simulink model "Pulse_Sweep_Model_Snapshot"  (R2026a)
settings: Solver=ode15s  StopTime=10  MaxStep=0.001  RelTol=1e-8  AbsTol=1e-10
model workspace (MAT data in the model file):
  K_lqr_controller = [-0.00284705017361 0.122689000645 -0.00232682606921 0.00886461536906]
  K_pp_controller = [-0.00262883953839 0.104642532618 -0.00218085328178 0.00778047678221]
  pid_ArmD = 0.00283510926632
  pid_ArmI = 0.0007
  pid_ArmP = 0.00184018767687
  pid_Kaw = 20
  pid_PendD = 0.00972559597776
  pid_PendP = 0.104642532618
  smiData.RigidTransform(1).translation = [-244.660692531 -37.8098812469 -477.156945201]
  smiData.RigidTransform(1).angle = 2.55760922614
  smiData.RigidTransform(1).axis = [0.300426658947 0.67440706052 0.674476789308]
  smiData.RigidTransform(1).ID = "B[modern conttrol_Pendulum .stp-1:-:modern conttrol_ horizontal_arm .stp-1]"
  smiData.RigidTransform(2).translation = [-247.634754981 -40.4847554626 -477.157635298]
  smiData.RigidTransform(2).angle = 2.55760922614
  smiData.RigidTransform(2).axis = [0.300426658947 0.67440706052 0.674476789308]
  smiData.RigidTransform(2).ID = "F[modern conttrol_Pendulum .stp-1:-:modern conttrol_ horizontal_arm .stp-1]"
  smiData.RigidTransform(3).translation = [-272.175879601 -62.5545266142 -447.163329111]
  smiData.RigidTransform(3).angle = 3.14152402451
  smiData.RigidTransform(3).axis = [-0.999999996374 2.92211836945e-09 -8.51568583922e-05]
  smiData.RigidTransform(3).ID = "B[modern conttrol_ horizontal_arm .stp-1:-:modern conttrol_ BASE .stp-1]"
  smiData.RigidTransform(4).translation = [-272.175879601 -62.5545266142 -447.163329111]
  smiData.RigidTransform(4).angle = 3.14152402451
  smiData.RigidTransform(4).axis = [-0.999999996374 2.92211836944e-09 -8.51568583922e-05]
  smiData.RigidTransform(4).ID = "F[modern conttrol_ horizontal_arm .stp-1:-:modern conttrol_ BASE .stp-1]"
  smiData.RigidTransform(5).translation = [-901.384854799 -324.852677228 2108.86942688]
  smiData.RigidTransform(5).angle = 2.09421753207
  smiData.RigidTransform(5).axis = [0.577330696727 -0.577330696727 0.577389412124]
  smiData.RigidTransform(5).ID = "RootGround[modern conttrol_ BASE .stp-1]"
  smiData.Solid(1).mass = 0.183317957018
  smiData.Solid(1).CoM = [-10.7361053602 -2.48129316166 -18.6438450111]
  smiData.Solid(1).MoI = [0.234552178635 0.234414857876 0.220551589316]
  smiData.Solid(1).PoI = [-0.000864428028976 -0.000962178736372 0.000630134655694]
  smiData.Solid(1).color = [0.745098039216 0.737254901961 0.729411764706]
  smiData.Solid(1).opacity = 1
  smiData.Solid(1).ID = "modern conttrol_ horizontal_arm .stp*:*Default"
  smiData.Solid(2).mass = 0.00722125286234
  smiData.Solid(2).CoM = [-8.92893482987 -1.82055355389 -18.2809598406]
  smiData.Solid(2).MoI = [0.0072083021969 0.0106803033814 0.00963261515156]
  smiData.Solid(2).PoI = [0.00327189358985 -0.00494008093961 0.00363251936408]
  smiData.Solid(2).color = [0.894117647059 0.894117647059 0.894117647059]
  smiData.Solid(2).opacity = 1
  smiData.Solid(2).ID = "modern conttrol_Pendulum .stp*:*Default"
  smiData.Solid(3).mass = 0.277142549471
  smiData.Solid(3).CoM = [-10.7265338957 -2.42898357651 -14.4295668435]
  smiData.Solid(3).MoI = [0.902926430859 0.896181432603 0.660496847328]
  smiData.Solid(3).PoI = [-0.0116443332078 0.00507741067153 0.00049862544881]
  smiData.Solid(3).color = [0.745098039216 0.737254901961 0.729411764706]
  smiData.Solid(3).opacity = 1
  smiData.Solid(3).ID = "modern conttrol_ BASE .stp*:*Default"
  smiData.RevoluteJoint(1).Rz.Pos = -7.13735250286e-12
  smiData.RevoluteJoint(1).ID = "[modern conttrol_Pendulum .stp-1:-:modern conttrol_ horizontal_arm .stp-1]"
  smiData.RevoluteJoint(2).Rz.Pos = -14.9000381004
  smiData.RevoluteJoint(2).ID = "[modern conttrol_ horizontal_arm .stp-1:-:modern conttrol_ BASE .stp-1]"
  tau_limit_sim = 0.01
  taue_controller = 6.71011527243e-16
  xe_controller = [0; 3.17402050778e-05; 0; 0]
undefined symbols (not defined in the file or in its folder): X, Y, Z
libraries: sm_lib x15, nesl_utility x6
settings Model: Creator=youss  LastModifiedBy=youss
settings ExplorerConfigSet: InternalSimMechanicsExplorerSettings=|
  | <ExplorerConfiguration>
  | 
  |   <canonicalview>planar_xy</canonicalview>
  | 
  |   <TilePanel>
  |     <TileInfo>
  |       <Tiles Columns="1" Count="1" Height="661" Rows="1" Width="1082">
  |         <Row Weight="1"/>
  |         <Column Weight="1"/>
  |         <Tile Height="1" Width="1" X="0" Y="0"/>
  |       </Tiles>
  |     </TileInfo>
  |     <SceneInfo>
  |       <SceneViewer>
  |         <IsThisViewStd>
  |           <IsStandardView>off</IsStandardView>
  |           <StandardViewName>Front</StandardViewName>
  |         </IsThisViewStd>
  |         <BGColor>
  |           <R>1</R>
  |           <G>1</G>
  |           <B>1</B>
  |           <A>1</A>
  |         </BGColor>
  |         <Camera>
  |           <DoPerspective>off</DoPerspective>
  |           <Position>
  |             <X>-0.83937932035154528</X>
  |             <Y>0.78777288036255699</Y>
  |             <Z>2.49476630807056</Z>
  |           </Position>
  |           <Center>
  |             <X>-0.83937932035154528</X>
  |             <Y>0.12962840465429493</Y>
  |             <Z>1.8366218323622983</Z>
  |           </Center>
  |           <Up>
  |             <X>0</X>
  |             <Y>0.70710678118654735</Y>
  |             <Z>-0.70710678118654768</Z>
  |           </Up>
  |           <XLim>0.13809857222982996</XLim>
  |           <YLim>0.13809857222982996</YLim>
  |           <ViewLimDist>0.01</ViewLimDist>
  |         </Camera>
  |       </SceneViewer>
  |     </SceneInfo>
  |   </TilePanel>
  | 
  |   <MechEditorPanel>
  |     <GfxPanelCameraMap/>
  |     <Cameras/>
  |     <VideoCreator>
  |       <IncludeTiles>All</IncludeTiles>
  |       <IncludeTime>on</IncludeTime>
  |       <IncludeWorldFrame>off</IncludeWorldFrame>
  |       <PlaybackSpeedRatio>1</PlaybackSpeedRatio>
  |       <FrameRate>30</FrameRate>
  |       <FrameSize>auto</FrameSize>
  |       <VideoFormat>UncompressedAVI</VideoFormat>
  |     </VideoCreator>
  |   </MechEditorPanel>
  | 
  |   <PlaybackSettings>
  |     <PlaybackSpeedFactor>1</PlaybackSpeedFactor>
  |   </PlaybackSettings>
  | 
  | </ExplorerConfiguration>

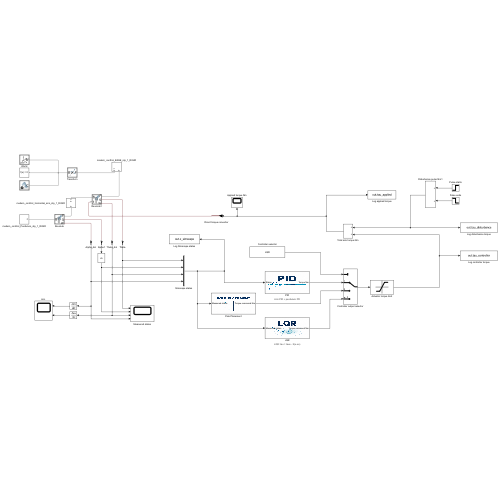
[thumbnail: Simulink's stored preview of the top-level diagram]
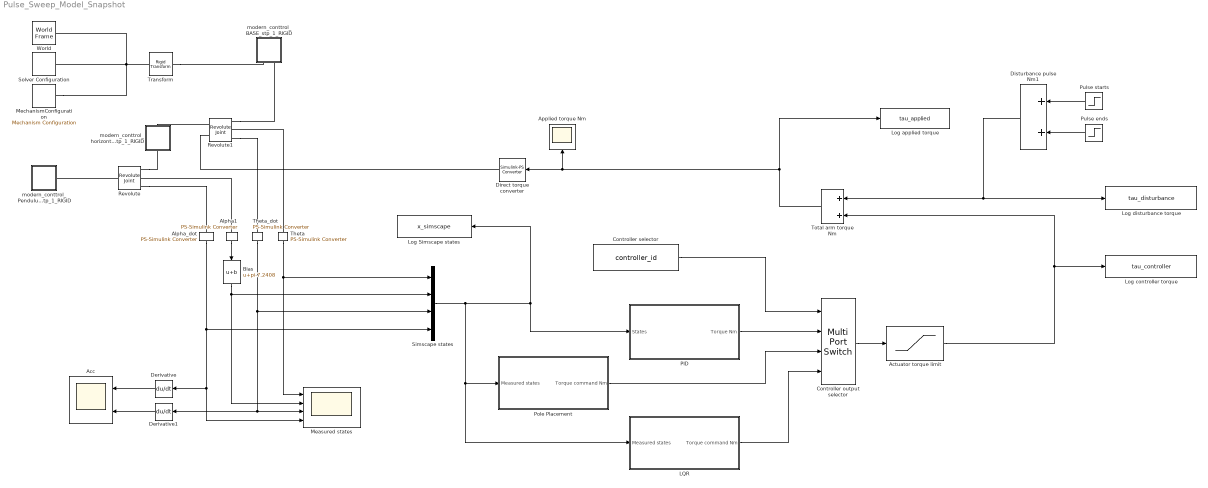
== system Pulse_Sweep_Model_Snapshot ==
  "Acc " : Scope  NumInputPorts=2
      settings: ActiveDisplayYMinimum=-146.28941148090837  ActiveDisplayYMaximum=145.24989573549755  YLabel=Arm
  Actuator torque limit : Saturate  UpperLimit=tau_limit_sim  LowerLimit=-tau_limit_sim
  Alpha1 : nesl_utility/PS-Simulink Converter  PhysicalDomain=network_engine_domain  SubClassName=ps_output  LeftPortType=input  RightPortType=output  PseudoPeriodic=off  Frequencies=[]  VectorFormat=inherit  Unit=rad  AffineConversion=off
  Alpha_dot : nesl_utility/PS-Simulink Converter  PhysicalDomain=network_engine_domain  SubClassName=ps_output  LeftPortType=input  RightPortType=output  PseudoPeriodic=off  Frequencies=[]  VectorFormat=inherit  Unit=rad/s  AffineConversion=off
  Applied torque Nm : Scope
      settings: Title=Total applied arm torque  ActiveDisplayYMinimum=-0.012433392383790797  ActiveDisplayYMaximum=0.014826694316528995  YLabel=N m
  Bias : Bias  Bias=pi-7.2408  SaturateOnIntegerOverflow=off
  Controller output selector : MultiPortSwitch  SaturateOnIntegerOverflow=off  InputSameDT=off
  Controller selector : Constant  Value=controller_id  SampleTime=0  mask{controller_choice=LQR}
      mask prompts: controller_choice "Controller"
      mask help: Choose the controller before simulation. PID and LQR are reserved until their gains are designed.
      mask init:
      | controller_id=find(strcmp(controller_choice,{'PID','Pole Placement','LQR'}));
      mask TypeOptions controller_choice: PID | Pole Placement | LQR
      mask Display: disp(controller_choice)
  Derivative : Derivative
  Derivative1 : Derivative
  Direct torque converter : nesl_utility/Simulink-PS Converter  PhysicalDomain=network_engine_domain  SubClassName=ps_input  LeftPortType=input  RightPortType=output  PseudoPeriodic=off  Frequencies=[]  NoiseDistribution=none  NoiseParameters=[]  Unit=N*m  AffineConversion=off  FilteringAndDerivatives=provide  SimscapeFilterOrder=1  InputFilterTimeConstant=0.001  UdotUserProvided=0
  Disturbance pulse Nm1 : Sum
  LQR : Subsystem  Description=Continuous four-state LQR using measured Multibody states. Shared actuator saturation remains outside the controller.
      settings: AttributesFormatString=LQR: tau = taue - K(x-xe)
      mask Display: image('ChatGPT Image Oct 27, 2026, 06_34_36 PM.png');
  Log Simscape states : ToWorkspace  VariableName=x_simscape  SaveFormat=Timeseries  SampleTime=-1
  Log applied torque : ToWorkspace  VariableName=tau_applied  SaveFormat=Timeseries  SampleTime=-1
  Log controller torque : ToWorkspace  VariableName=tau_controller  SaveFormat=Timeseries  SampleTime=-1
  Log disturbance torque : ToWorkspace  VariableName=tau_disturbance  SaveFormat=Timeseries  SampleTime=-1
  Measured states : Scope  NumInputPorts=4
      settings: Title=Arm angle - theta  ActiveDisplayYMinimum=-0.33373854489322996  ActiveDisplayYMaximum=0.16467513422765392  YLabel=rad
  MechanismConfiguration : sm_lib/Utilities/Mechanism Configuration  UniformGravity=Constant  GravityVector=[0 -9.81 0]  GravityVectorUnits=m/s^2  LinearizationDelta=0.001  JointModeTransitionNonlinearIterations=2
  PID : Subsystem  Description=Simple P/I/D paths. Select controller before each fresh run. No inactive tracking or live switching.
      settings: AttributesFormatString=Arm PID + pendulum PD
      mask Display: image('ChatGPT Image Oct 27, 2026, 06_33_53 PM.png');
  Pole Placement : Subsystem
      mask Display: image('ChatGPT Image Oct 27, 2026, 06_34_26 PM.png');
  Pulse ends : Step  Time=1.05  FinalValue=-0.01  SampleTime=0
  Pulse starts : Step  FinalValue=0.01  SampleTime=0
  Revolute : sm_lib/Joints/Revolute Joint  JointMode=Normal  CompositeWrenchDir=FollowerOnBase  CompositeWrenchFrame=BaseFrame  SenseConstraintForce=off  SenseConstraintTorque=off  SenseTotalForce=off  SenseTotalTorque=off  PositionTargetSpecify=on  PositionTargetPriority=High  PositionTargetValue=7.2408 -pi  PositionTargetValueUnits=rad  VelocityTargetSpecify=on  VelocityTargetPriority=High  VelocityTargetValue=0  VelocityTargetValueUnits=rad/s  EquilibriumPosition=0  EquilibriumPositionUnits=deg  SpringStiffness=0  SpringStiffnessUnits=N*m/deg  DampingCoefficient=5.5e-7  DampingCoefficientUnits=N*m/(deg/s)  LowerLimitSpecify=off  LowerLimitBound=-90  LowerLimitBoundUnits=deg  LowerLimitStiffness=1e4  LowerLimitStiffnessUnits=N*m/deg  LowerLimitDamping=10  LowerLimitDampingUnits=N*m/(deg/s)  LowerLimitTransitionRegionWidth=0.1  LowerLimitTransitionRegionWidthUnits=deg  UpperLimitSpecify=off  UpperLimitBound=90  UpperLimitBoundUnits=deg  UpperLimitStiffness=1e4  UpperLimitStiffnessUnits=N*m/deg  UpperLimitDamping=10  UpperLimitDampingUnits=N*m/(deg/s)  UpperLimitTransitionRegionWidth=0.1  UpperLimitTransitionRegionWidthUnits=deg  TorqueActuationMode=NoTorque  MotionActuationMode=ComputedMotion  SensePosition=on  SenseVelocity=on  SenseAcceleration=off  SenseTorqueForce=off  SenseLowerLimitTorqueForce=off  SenseUpperLimitTorqueForce=off
  Revolute1 : sm_lib/Joints/Revolute Joint  JointMode=Normal  CompositeWrenchDir=FollowerOnBase  CompositeWrenchFrame=BaseFrame  SenseConstraintForce=off  SenseConstraintTorque=off  SenseTotalForce=off  SenseTotalTorque=off  PositionTargetSpecify=off  PositionTargetPriority=High  PositionTargetValue=0  PositionTargetValueUnits=deg  VelocityTargetSpecify=off  VelocityTargetPriority=High  VelocityTargetValue=0  VelocityTargetValueUnits=deg/s  EquilibriumPosition=0  EquilibriumPositionUnits=deg  SpringStiffness=0  SpringStiffnessUnits=N*m/deg  DampingCoefficient=1e-5  DampingCoefficientUnits=N*m/(deg/s)  LowerLimitSpecify=off  LowerLimitBound=-90  LowerLimitBoundUnits=deg  LowerLimitStiffness=1e4  LowerLimitStiffnessUnits=N*m/deg  LowerLimitDamping=10  LowerLimitDampingUnits=N*m/(deg/s)  LowerLimitTransitionRegionWidth=0.1  LowerLimitTransitionRegionWidthUnits=deg  UpperLimitSpecify=off  UpperLimitBound=90  UpperLimitBoundUnits=deg  UpperLimitStiffness=1e4  UpperLimitStiffnessUnits=N*m/deg  UpperLimitDamping=10  UpperLimitDampingUnits=N*m/(deg/s)  UpperLimitTransitionRegionWidth=0.1  UpperLimitTransitionRegionWidthUnits=deg  TorqueActuationMode=InputTorque  MotionActuationMode=ComputedMotion  SensePosition=on  SenseVelocity=on  SenseAcceleration=off  SenseTorqueForce=off  SenseLowerLimitTorqueForce=off  SenseUpperLimitTorqueForce=off
  Simscape states : Mux
  Solver Configuration : nesl_utility/Solver Configuration  PhysicalDomain=network_engine_domain  SubClassName=solver  LeftPortType=input  RightPortType=generic  Tones=[]  Harmonics=[]  SimulateNoise=off  Profile=off  UseLocalSampling=off  EnableSwitchedLinearOptims=on  FrequencyDomain=off  UseCCode=off  RelTol=0.001  AbsTol=0.001  MinStep=1e-09  ToWorkspace=off  RevertToSquareIcSolve=off  NumHomotopyIterations=100  PhasorMode=off  PhasorModeNumHarmonics=1  ConsistencySolver=NEWTON_XTOL_AFTER_FTOL  CanonicalOrdering=CANONICAL  OptimizeIntermediates=OPTIMIZED  IndexReductionMethod=DerivativeReplacement  DoDC=off  ResidualTolerance=1e-09  ConsistencyTolSource=GLOBAL  ConsistencyAbsTol=0.001  ConsistencyRelTol=0.001  ConsistencyTolFactor=0.001  UseLocalSolver=off  LocalSolverChoice=NE_BACKWARD_EULER_ADVANCER  ResolveIndetEquations=on  FunctionEvalNumThread=1  LocalSolverSampleTime=0.001  DoFixedCost=off  MaxNonlinIter=3  MaxModeIter=2  ComputeImpulses=off  ImpulseIterations=2  LinearAlgebra=auto  LinearAlgebraNumThread=0  EquationFormulation=NE_TIME_EF  DelaysMemoryBudget=1024  AutomaticFiltering=on  FilteringTimeConstant=0.001  PartitionStorageMethod=AS_NEEDED  PartitionMemoryBudget=1024  PartitionMethod=ROBUST  MultibodyUseLocalSolver=off  MultibodyLocalSolverChoice=ODE1  MultibodyLocalSolverSampleTime=0.001
  Theta : nesl_utility/PS-Simulink Converter  PhysicalDomain=network_engine_domain  SubClassName=ps_output  LeftPortType=input  RightPortType=output  PseudoPeriodic=off  Frequencies=[]  VectorFormat=inherit  Unit=rad  AffineConversion=off
  Theta_dot : nesl_utility/PS-Simulink Converter  PhysicalDomain=network_engine_domain  SubClassName=ps_output  LeftPortType=input  RightPortType=output  PseudoPeriodic=off  Frequencies=[]  VectorFormat=inherit  Unit=rad/s  AffineConversion=off
  Total arm torque Nm : Sum
  Transform : sm_lib/Frames and Transforms/Rigid Transform  RotationMethod=ArbitraryAxis  FollAlignAxisA=+X  BaseAlignAxisA=+Y  FollAlignAxisB=+Y  BaseAlignAxisB=+Z  RotationStandardAxis=+Z  RotationAngle=smiData.RigidTransform(5).angle  RotationAngleUnits=rad  RotationArbitraryAxis=smiData.RigidTransform(5).axis  RotationSequenceAxes=FollowerAxes  RotationSequence=XYX  RotationSequenceAngles=[0 0 0]  RotationSequenceAnglesUnits=deg  RotationMatrix=[1 0 0;0 1 0;0 0 1]  Quaternion=[1 0 0 0]  TranslationMethod=Cartesian  TranslationCartesianOffset=smiData.RigidTransform(5).translation  TranslationCartesianOffsetUnits=mm  TranslationStandardAxis=+Z  TranslationStandardOffset=0  TranslationStandardOffsetUnits=m  TranslationROffset=0  TranslationROffsetUnits=m  TranslationThetaOffset=0  TranslationThetaOffsetUnits=deg  TranslationZOffset=0  TranslationZOffsetUnits=m
  World : sm_lib/Frames and Transforms/World Frame
  modern_conttrol_BASE_stp_1_RIGID : Subsystem
  modern_conttrol_Pendulum_stp_1_RIGID : Subsystem
  modern_conttrol_horizontal_arm_stp_1_RIGID : Subsystem
  wires:
  Theta/1 -> Simscape states/1, Measured states/1
  Bias/1 -> Simscape states/2, Measured states/2
  Alpha1/1 -> Bias/1
  Simscape states/1 -> PID/1(States), Log Simscape states/1, LQR/1(Measured states), Pole Placement/1(Measured states)
  Total arm torque Nm/1 -> Applied torque Nm/1, Direct torque converter/1, Log applied torque/1
  Actuator torque limit/1 -> Total arm torque Nm/2, Log controller torque/1
  Controller selector/1 -> Controller output selector/1
  Pole Placement/1(Torque command Nm) -> Controller output selector/3
  LQR/1(Torque command Nm) -> Controller output selector/4
  Controller output selector/1 -> Actuator torque limit/1
  PID/1(Torque Nm) -> Controller output selector/2
  Derivative1/1 -> "Acc "/2
  Alpha_dot/1 -> Simscape states/4, Derivative/1, Measured states/4
  Derivative/1 -> "Acc "/1
  Theta_dot/1 -> Simscape states/3, Measured states/3, Derivative1/1
  Pulse ends/1 -> Disturbance pulse Nm1/2
  Pulse starts/1 -> Disturbance pulse Nm1/1
  Disturbance pulse Nm1/1 -> Log disturbance torque/1, Total arm torque Nm/1
  connections:
  MechanismConfiguration/RConn1 -- Transform/LConn1 -- Solver Configuration/RConn1 -- World/RConn1
  Revolute/LConn1 -- modern_conttrol_Pendulum_stp_1_RIGID/RConn1
  Revolute/RConn1 -- modern_conttrol_horizontal_arm_stp_1_RIGID/LConn1
  Revolute1/LConn1 -- modern_conttrol_horizontal_arm_stp_1_RIGID/RConn1
  Revolute1/RConn1 -- modern_conttrol_BASE_stp_1_RIGID/LConn2
  Transform/RConn1 -- modern_conttrol_BASE_stp_1_RIGID/LConn1
  Theta/LConn1 -- Revolute1/RConn2
  Revolute/RConn3 -- Alpha_dot/LConn1
  Alpha1/LConn1 -- Revolute/RConn2
  Revolute1/RConn3 -- Theta_dot/LConn1
  Direct torque converter/RConn1 -- Revolute1/LConn2

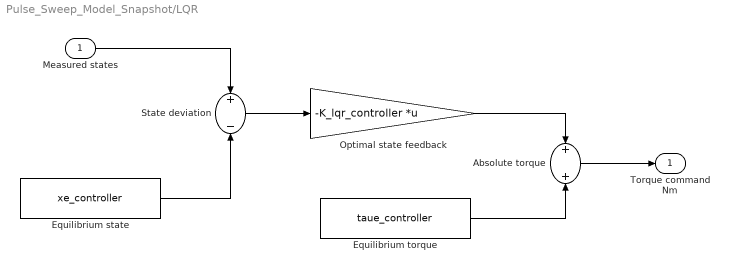
== system Pulse_Sweep_Model_Snapshot/LQR ==
  Measured states : Inport
  Absolute torque : Sum
  Equilibrium state : Constant  Value=xe_controller
  Equilibrium torque : Constant  Value=taue_controller
  Optimal state feedback : Gain  Gain=-K_lqr_controller  Multiplication=Matrix(K*u)
  State deviation : Sum  Inputs=+-
  Torque command Nm : Outport
  wires:
  Measured states/1 -> State deviation/1
  Equilibrium state/1 -> State deviation/2
  State deviation/1 -> Optimal state feedback/1
  Optimal state feedback/1 -> Absolute torque/1
  Equilibrium torque/1 -> Absolute torque/2
  Absolute torque/1 -> Torque command Nm/1

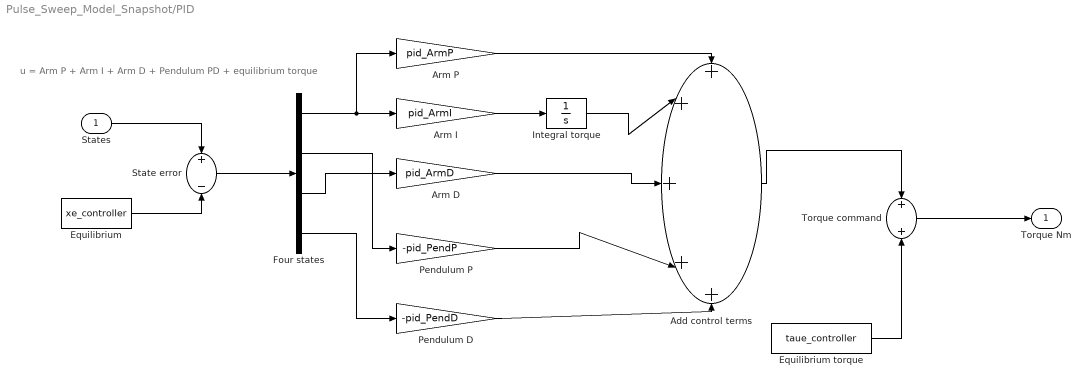
== system Pulse_Sweep_Model_Snapshot/PID ==
  note: u = Arm P + Arm I + Arm D + Pendulum PD + equilibrium torque
  States : Inport
  Add control terms : Sum  Inputs=+++++
  Arm D : Gain  Gain=pid_ArmD
  Arm I : Gain  Gain=pid_ArmI
  Arm P : Gain  Gain=pid_ArmP
  Equilibrium : Constant  Value=xe_controller
  Equilibrium torque : Constant  Value=taue_controller
  Four states : Demux
  Integral torque : Integrator  LimitOutput=on  UpperSaturationLimit=0.002  LowerSaturationLimit=-0.002
  Pendulum D : Gain  Gain=-pid_PendD
  Pendulum P : Gain  Gain=-pid_PendP
  State error : Sum  Inputs=+-
  Torque command : Sum
  Torque Nm : Outport
  wires:
  States/1 -> State error/1
  Equilibrium/1 -> State error/2
  State error/1 -> Four states/1
  Four states/1 -> Arm P/1, Arm I/1
  Four states/3 -> Arm D/1
  Four states/2 -> Pendulum P/1
  Four states/4 -> Pendulum D/1
  Arm I/1 -> Integral torque/1
  Arm P/1 -> Add control terms/1
  Integral torque/1 -> Add control terms/2
  Arm D/1 -> Add control terms/3
  Pendulum P/1 -> Add control terms/4
  Pendulum D/1 -> Add control terms/5
  Add control terms/1 -> Torque command/1
  Equilibrium torque/1 -> Torque command/2
  Torque command/1 -> Torque Nm/1

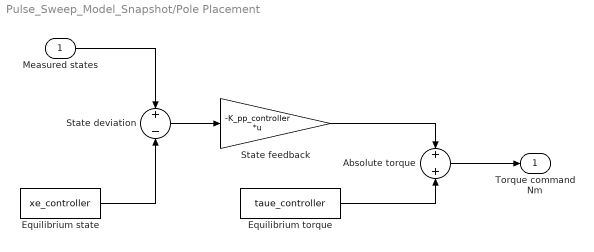
== system Pulse_Sweep_Model_Snapshot/Pole Placement ==
  Measured states : Inport
  Absolute torque : Sum
  Equilibrium state : Constant  Value=xe_controller
  Equilibrium torque : Constant  Value=taue_controller
  State deviation : Sum  Inputs=+-
  State feedback : Gain  Gain=-K_pp_controller  Multiplication=Matrix(K*u)
  Torque command Nm : Outport
  wires:
  Measured states/1 -> State deviation/1
  Equilibrium state/1 -> State deviation/2
  State deviation/1 -> State feedback/1
  State feedback/1 -> Absolute torque/1
  Equilibrium torque/1 -> Absolute torque/2
  Absolute torque/1 -> Torque command Nm/1

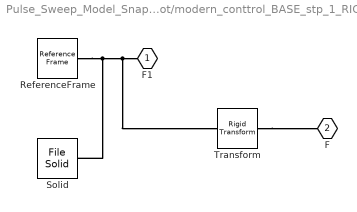
== system Pulse_Sweep_Model_Snapshot/modern_conttrol_BASE_stp_1_RIGID ==
  ReferenceFrame : sm_lib/Frames and Transforms/Reference Frame
  Solid : sm_lib/Body Elements/File Solid  ExtGeomFileName=modern conttrol_ BASE .stp_Default_sldprt.STEP  UnitType=FromFile  ExtGeomFileUnits=m  StepReaderType=HEX  ExportConvexHullGeometry=off  InertiaType=Custom  BasedOnType=DensityFromFile  Density=1000  DensityUnits=kg/m^3  Mass=smiData.Solid(3).mass  MassUnits=kg  CenterOfMass=smiData.Solid(3).CoM  CenterOfMassUnits=in  MomentsOfInertia=smiData.Solid(3).MoI  MomentsOfInertiaUnits=kg*in^2  ProductsOfInertia=smiData.Solid(3).PoI  ProductsOfInertiaUnits=kg*in^2  GraphicType=FromGeometry  MarkerShape=Sphere  MarkerSize=10  GraphicVisPropType=SimpleVisualProperties  GraphicDiffuseColor=[0.8745 0 0]  GraphicOpacity=smiData.Solid(3).opacity  GraphicSpecularColor=[0.5 0.5 0.5 1.0]  GraphicAmbientColor=[0.15 0.15 0.15 1.0]  GraphicEmissiveColor=[0.0 0.0 0.0 1.0]  GraphicShininess=75  DoExposeReferenceFrame=on  SerializedFrames=<Frames/>
  Transform : sm_lib/Frames and Transforms/Rigid Transform  RotationMethod=ArbitraryAxis  FollAlignAxisA=+X  BaseAlignAxisA=+Y  FollAlignAxisB=+Y  BaseAlignAxisB=+Z  RotationStandardAxis=+Z  RotationAngle=smiData.RigidTransform(4).angle  RotationAngleUnits=rad  RotationArbitraryAxis=smiData.RigidTransform(4).axis  RotationSequenceAxes=FollowerAxes  RotationSequence=XYX  RotationSequenceAngles=[0 0 0]  RotationSequenceAnglesUnits=deg  RotationMatrix=[1 0 0;0 1 0;0 0 1]  Quaternion=[1 0 0 0]  TranslationMethod=Cartesian  TranslationCartesianOffset=smiData.RigidTransform(4).translation  TranslationCartesianOffsetUnits=mm  TranslationStandardAxis=+Z  TranslationStandardOffset=0  TranslationStandardOffsetUnits=m  TranslationROffset=0  TranslationROffsetUnits=m  TranslationThetaOffset=0  TranslationThetaOffsetUnits=deg  TranslationZOffset=0  TranslationZOffsetUnits=m
  F1 : PMIOPort  Side=Left
  F : PMIOPort  Port=2  Side=Left
  connections:
  Solid/RConn1 -- ReferenceFrame/RConn1 -- Transform/LConn1 -- F1/RConn1
  Transform/RConn1 -- F/RConn1

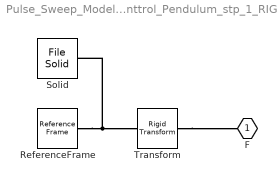
== system Pulse_Sweep_Model_Snapshot/modern_conttrol_Pendulum_stp_1_RIGID ==
  ReferenceFrame : sm_lib/Frames and Transforms/Reference Frame
  Solid : sm_lib/Body Elements/File Solid  ExtGeomFileName=modern conttrol_Pendulum .stp_Default_sldprt.STEP  UnitType=FromFile  ExtGeomFileUnits=m  StepReaderType=HEX  ExportConvexHullGeometry=off  InertiaType=Custom  BasedOnType=DensityFromFile  Density=1000  DensityUnits=kg/m^3  Mass=smiData.Solid(2).mass  MassUnits=kg  CenterOfMass=smiData.Solid(2).CoM  CenterOfMassUnits=in  MomentsOfInertia=smiData.Solid(2).MoI  MomentsOfInertiaUnits=kg*in^2  ProductsOfInertia=smiData.Solid(2).PoI  ProductsOfInertiaUnits=kg*in^2  GraphicType=FromGeometry  MarkerShape=Sphere  MarkerSize=10  GraphicVisPropType=SimpleVisualProperties  GraphicDiffuseColor=[0 0.5569 0.8353]  GraphicOpacity=smiData.Solid(2).opacity  GraphicSpecularColor=[0.5 0.5 0.5 1.0]  GraphicAmbientColor=[0.15 0.15 0.15 1.0]  GraphicEmissiveColor=[0.0 0.0 0.0 1.0]  GraphicShininess=75  DoExposeReferenceFrame=on  SerializedFrames=<Frames/>
  Transform : sm_lib/Frames and Transforms/Rigid Transform  RotationMethod=ArbitraryAxis  FollAlignAxisA=+X  BaseAlignAxisA=+Y  FollAlignAxisB=+Y  BaseAlignAxisB=+Z  RotationStandardAxis=+Z  RotationAngle=smiData.RigidTransform(1).angle  RotationAngleUnits=rad  RotationArbitraryAxis=smiData.RigidTransform(1).axis  RotationSequenceAxes=FollowerAxes  RotationSequence=XYX  RotationSequenceAngles=[0 0 0]  RotationSequenceAnglesUnits=deg  RotationMatrix=[1 0 0;0 1 0;0 0 1]  Quaternion=[1 0 0 0]  TranslationMethod=Cartesian  TranslationCartesianOffset=smiData.RigidTransform(1).translation  TranslationCartesianOffsetUnits=mm  TranslationStandardAxis=+Z  TranslationStandardOffset=0  TranslationStandardOffsetUnits=m  TranslationROffset=0  TranslationROffsetUnits=m  TranslationThetaOffset=0  TranslationThetaOffsetUnits=deg  TranslationZOffset=0  TranslationZOffsetUnits=m
  F : PMIOPort  Side=Right
  connections:
  Solid/RConn1 -- ReferenceFrame/RConn1 -- Transform/LConn1
  Transform/RConn1 -- F/RConn1

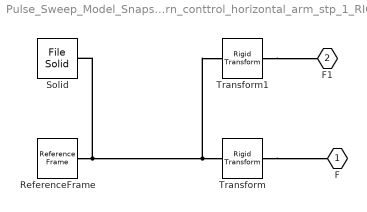
== system Pulse_Sweep_Model_Snapshot/modern_conttrol_horizontal_arm_stp_1_RIGID ==
  ReferenceFrame : sm_lib/Frames and Transforms/Reference Frame
  Solid : sm_lib/Body Elements/File Solid  ExtGeomFileName=modern conttrol_ horizontal_arm .stp_Default_sldprt.STEP  UnitType=FromFile  ExtGeomFileUnits=m  StepReaderType=HEX  ExportConvexHullGeometry=off  InertiaType=Custom  BasedOnType=DensityFromFile  Density=1000  DensityUnits=kg/m^3  Mass=smiData.Solid(1).mass  MassUnits=kg  CenterOfMass=smiData.Solid(1).CoM  CenterOfMassUnits=in  MomentsOfInertia=smiData.Solid(1).MoI  MomentsOfInertiaUnits=kg*in^2  ProductsOfInertia=smiData.Solid(1).PoI  ProductsOfInertiaUnits=kg*in^2  GraphicType=FromGeometry  MarkerShape=Sphere  MarkerSize=10  GraphicVisPropType=SimpleVisualProperties  GraphicDiffuseColor=[0.298 0.298 0.298]  GraphicOpacity=smiData.Solid(1).opacity  GraphicSpecularColor=[0.5 0.5 0.5 1.0]  GraphicAmbientColor=[0.15 0.15 0.15 1.0]  GraphicEmissiveColor=[0.0 0.0 0.0 1.0]  GraphicShininess=75  DoExposeReferenceFrame=on  SerializedFrames=<Frames/>
  Transform : sm_lib/Frames and Transforms/Rigid Transform  RotationMethod=ArbitraryAxis  FollAlignAxisA=+X  BaseAlignAxisA=+Y  FollAlignAxisB=+Y  BaseAlignAxisB=+Z  RotationStandardAxis=+Z  RotationAngle=smiData.RigidTransform(2).angle  RotationAngleUnits=rad  RotationArbitraryAxis=smiData.RigidTransform(2).axis  RotationSequenceAxes=FollowerAxes  RotationSequence=XYX  RotationSequenceAngles=[0 0 0]  RotationSequenceAnglesUnits=deg  RotationMatrix=[1 0 0;0 1 0;0 0 1]  Quaternion=[1 0 0 0]  TranslationMethod=Cartesian  TranslationCartesianOffset=smiData.RigidTransform(2).translation  TranslationCartesianOffsetUnits=mm  TranslationStandardAxis=+Z  TranslationStandardOffset=0  TranslationStandardOffsetUnits=m  TranslationROffset=0  TranslationROffsetUnits=m  TranslationThetaOffset=0  TranslationThetaOffsetUnits=deg  TranslationZOffset=0  TranslationZOffsetUnits=m
  Transform1 : sm_lib/Frames and Transforms/Rigid Transform  RotationMethod=ArbitraryAxis  FollAlignAxisA=+X  BaseAlignAxisA=+Y  FollAlignAxisB=+Y  BaseAlignAxisB=+Z  RotationStandardAxis=+Z  RotationAngle=smiData.RigidTransform(3).angle  RotationAngleUnits=rad  RotationArbitraryAxis=smiData.RigidTransform(3).axis  RotationSequenceAxes=FollowerAxes  RotationSequence=XYX  RotationSequenceAngles=[0 0 0]  RotationSequenceAnglesUnits=deg  RotationMatrix=[1 0 0;0 1 0;0 0 1]  Quaternion=[1 0 0 0]  TranslationMethod=Cartesian  TranslationCartesianOffset=smiData.RigidTransform(3).translation  TranslationCartesianOffsetUnits=mm  TranslationStandardAxis=+Z  TranslationStandardOffset=0  TranslationStandardOffsetUnits=m  TranslationROffset=0  TranslationROffsetUnits=m  TranslationThetaOffset=0  TranslationThetaOffsetUnits=deg  TranslationZOffset=0  TranslationZOffsetUnits=m
  F : PMIOPort  Side=Left
  F1 : PMIOPort  Port=2  Side=Right
  connections:
  Solid/RConn1 -- ReferenceFrame/RConn1 -- Transform/LConn1 -- Transform1/LConn1
  Transform/RConn1 -- F/RConn1
  Transform1/RConn1 -- F1/RConn1
